simulink model "Fixed_Base_Plant"  (R2026b)
settings: Solver=VariableStepAuto
undefined symbols (not defined in the file): fractalcoef, X, Y, Z
libraries: sm_lib x16, nesl_utility x9, Simulation_Blocks x2, simulink_extras x1, mspsensorlib x1
settings Model: Creator=Janelyn Anderson  LastModifiedBy=Janelyn Anderson

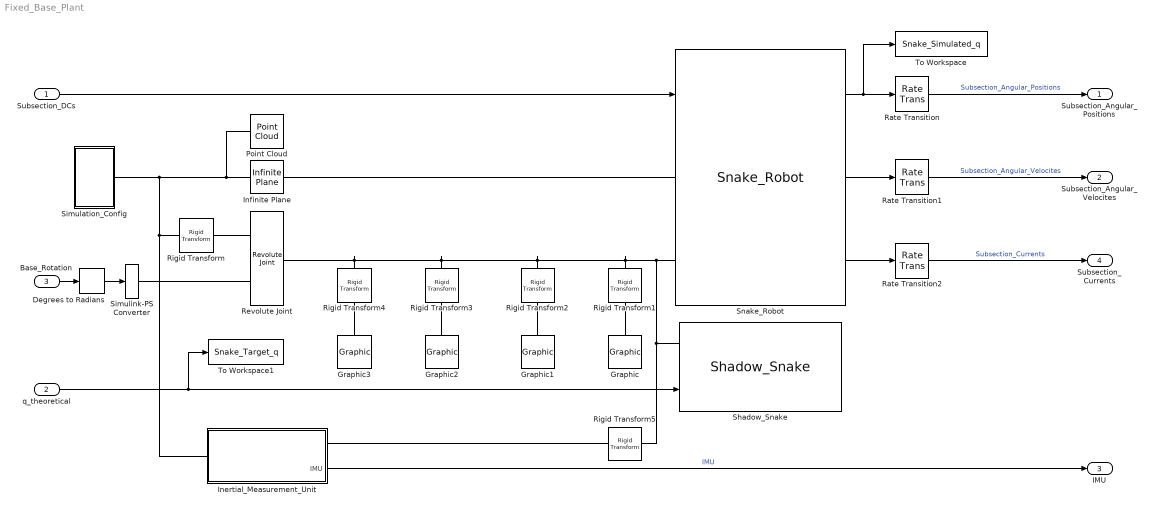
== system Fixed_Base_Plant ==
  Subsection_DCs : Inport
  q_theoretical : Inport  Port=2
  Base_Rotation : Inport  Port=3
  Degrees to Radians : simulink_extras/Transformations/Degrees to Radians
  Graphic : sm_lib/Body Elements/Graphic  GraphicType=Marker  MarkerShape=Sphere  MarkerSize=10  GraphicVisPropType=SimpleVisualProperties  GraphicDiffuseColor=[1 1 0]  GraphicOpacity=1  GraphicSpecularColor=[0.5 0.5 0.5 1.0]  GraphicAmbientColor=[0.15 0.15 0.15 1.0]  GraphicEmissiveColor=[0.0 0.0 0.0 1.0]  GraphicShininess=75
  Graphic1 : sm_lib/Body Elements/Graphic  GraphicType=Marker  MarkerShape=Sphere  MarkerSize=10  GraphicVisPropType=SimpleVisualProperties  GraphicDiffuseColor=[0 1 0]  GraphicOpacity=1  GraphicSpecularColor=[0.5 0.5 0.5 1.0]  GraphicAmbientColor=[0.15 0.15 0.15 1.0]  GraphicEmissiveColor=[0.0 0.0 0.0 1.0]  GraphicShininess=75
  Graphic2 : sm_lib/Body Elements/Graphic  GraphicType=Marker  MarkerShape=Sphere  MarkerSize=10  GraphicVisPropType=SimpleVisualProperties  GraphicDiffuseColor=[1 0 0]  GraphicOpacity=1  GraphicSpecularColor=[0.5 0.5 0.5 1.0]  GraphicAmbientColor=[0.15 0.15 0.15 1.0]  GraphicEmissiveColor=[0.0 0.0 0.0 1.0]  GraphicShininess=75
  Graphic3 : sm_lib/Body Elements/Graphic  GraphicType=Marker  MarkerShape=Sphere  MarkerSize=10  GraphicVisPropType=SimpleVisualProperties  GraphicDiffuseColor=[0 0 1]  GraphicOpacity=1  GraphicSpecularColor=[0.5 0.5 0.5 1.0]  GraphicAmbientColor=[0.15 0.15 0.15 1.0]  GraphicEmissiveColor=[0.0 0.0 0.0 1.0]  GraphicShininess=75
  Inertial_Measurement_Unit : Subsystem
      settings: PortSchema="{\"entries\":[{\"content\":{\"sides\":[{\"content\":{\"connectorIds\":[\"LConn1\"]},\"type\":\"ConnectorPlacement.EquallySpacedRectSide\",\"uuid\":\"83640582-12e8-48aa-a086-d986329aaf09\"},{\"content\":{\"connectorIds\":[\"RConn1\",\"Out1\"],\"side\":\"RIGHT\"},\"type\":\"ConnectorPlacement.EquallySpacedRectSide\",\"uuid\":\"2d285237-615f-43bd-9bcd-fec2f137a93b\"},{\"content\":{\"side\":\"TOP\"},\"type\":\"ConnectorPlacement.EquallySpacedRectSide\",\"uuid\":\"9a803d3e-15ac-4be1-bdbe-8bb20f8175ea\"}]},\"type\":\"ConnectorPlacement.EquallySpacedConnector\",\"uuid\":\"2b15680b-56f3-4ae6-a253-9b33d5e19e84\"}],\"packageUris\":[\"http://schema.mathworks.com/mf0/Connector/R2020b\"],\"version\":\"1.0\"}"
  Infinite Plane : sm_lib/Curves and Surfaces/Infinite Plane  GraphicType=Rectangle  GraphicPlaneWidth=2  GraphicPlaneWidthUnits=m  GraphicPlaneHeight=2  GraphicPlaneHeightUnits=m  GraphicVisPropType=AdvancedVisualProperties  GraphicDiffuseColor=[0.5 0.5 0.5]  GraphicOpacity=1  GraphicSpecularColor=[0.5 0.5 0.5 1.0]  GraphicAmbientColor=[0.15 0.15 0.15 1.0]  GraphicEmissiveColor=[0.0 0.0 0.0 1.0]  GraphicShininess=60
  Point Cloud : sm_lib/Curves and Surfaces/Point Cloud  CoordinatesMatrix=floorGrid  CoordinatesMatrixUnits=m  GraphicType=MarkerCloud  GraphicSphereRadius=1e-2  GraphicSphereRadiusUnits=m  GraphicVisPropType=SimpleVisualProperties  GraphicDiffuseColor=[0.3451 0.3333 0.6863]  GraphicOpacity=0.5  GraphicSpecularColor=[0.5 0.5 0.5 1.0]  GraphicAmbientColor=[0.15 0.15 0.15 1.0]  GraphicEmissiveColor=[0.0 0.0 0.0 1.0]  GraphicShininess=75
  Rate Transition : RateTransition  OutPortSampleTime=1/50
  Rate Transition1 : RateTransition  OutPortSampleTime=1/50
  Rate Transition2 : RateTransition  OutPortSampleTime=1/50
  Revolute Joint : sm_lib/Joints/Revolute Joint  JointMode=Normal  CompositeWrenchDir=FollowerOnBase  CompositeWrenchFrame=BaseFrame  SenseConstraintForce=off  SenseConstraintTorque=off  SenseTotalForce=off  SenseTotalTorque=off  PositionTargetSpecify=off  PositionTargetPriority=High  PositionTargetValue=0  PositionTargetValueUnits=deg  VelocityTargetSpecify=off  VelocityTargetPriority=High  VelocityTargetValue=0  VelocityTargetValueUnits=deg/s  EquilibriumPosition=0  EquilibriumPositionUnits=deg  SpringStiffness=0  SpringStiffnessUnits=N*m/deg  DampingCoefficient=0  DampingCoefficientUnits=N*m/(deg/s)  LowerLimitSpecify=on  LowerLimitBound=-90  LowerLimitBoundUnits=deg  LowerLimitStiffness=1e4  LowerLimitStiffnessUnits=N*m/deg  LowerLimitDamping=10  LowerLimitDampingUnits=N*m/(deg/s)  LowerLimitTransitionRegionWidth=0.1  LowerLimitTransitionRegionWidthUnits=deg  UpperLimitSpecify=on  UpperLimitBound=90  UpperLimitBoundUnits=deg  UpperLimitStiffness=1e4  UpperLimitStiffnessUnits=N*m/deg  UpperLimitDamping=10  UpperLimitDampingUnits=N*m/(deg/s)  UpperLimitTransitionRegionWidth=0.1  UpperLimitTransitionRegionWidthUnits=deg  TorqueActuationMode=ComputedTorque  MotionActuationMode=InputMotion  SensePosition=off  SenseVelocity=off  SenseAcceleration=off  SenseTorqueForce=off  SenseLowerLimitTorqueForce=off  SenseUpperLimitTorqueForce=off
  Rigid Transform : sm_lib/Frames and Transforms/Rigid Transform  RotationMethod=RotationSequence  FollAlignAxisA=+X  BaseAlignAxisA=+Y  FollAlignAxisB=+Y  BaseAlignAxisB=+Z  RotationStandardAxis=+X  RotationAngle=90  RotationAngleUnits=deg  RotationArbitraryAxis=[0 0 1]  RotationSequenceAxes=FollowerAxes  RotationSequence=XZX  RotationSequenceAngles=[90 0 0]  RotationSequenceAnglesUnits=deg  RotationMatrix=[1 0 0;0 1 0;0 0 1]  Quaternion=[1 0 0 0]  TranslationMethod=Cartesian  TranslationCartesianOffset=[0 0 20]  TranslationCartesianOffsetUnits=in  TranslationStandardAxis=+Z  TranslationStandardOffset=0  TranslationStandardOffsetUnits=m  TranslationROffset=0  TranslationROffsetUnits=m  TranslationThetaOffset=0  TranslationThetaOffsetUnits=deg  TranslationZOffset=0  TranslationZOffsetUnits=m
  Rigid Transform1 : sm_lib/Frames and Transforms/Rigid Transform  RotationMethod=StandardAxis  FollAlignAxisA=+X  BaseAlignAxisA=+Y  FollAlignAxisB=+Y  BaseAlignAxisB=+Z  RotationStandardAxis=+Z  RotationAngle=0  RotationAngleUnits=deg  RotationArbitraryAxis=[0 0 1]  RotationSequenceAxes=FollowerAxes  RotationSequence=XYX  RotationSequenceAngles=[0 0 0]  RotationSequenceAnglesUnits=deg  RotationMatrix=[1 0 0;0 1 0;0 0 1]  Quaternion=[1 0 0 0]  TranslationMethod=StandardAxis  TranslationCartesianOffset=[0 0 0]  TranslationCartesianOffsetUnits=m  TranslationStandardAxis=-X  TranslationStandardOffset=1.5  TranslationStandardOffsetUnits=ft  TranslationROffset=0  TranslationROffsetUnits=m  TranslationThetaOffset=0  TranslationThetaOffsetUnits=deg  TranslationZOffset=0  TranslationZOffsetUnits=m
  Rigid Transform2 : sm_lib/Frames and Transforms/Rigid Transform  RotationMethod=StandardAxis  FollAlignAxisA=+X  BaseAlignAxisA=+Y  FollAlignAxisB=+Y  BaseAlignAxisB=+Z  RotationStandardAxis=+Z  RotationAngle=90  RotationAngleUnits=deg  RotationArbitraryAxis=[0 0 1]  RotationSequenceAxes=FollowerAxes  RotationSequence=XYX  RotationSequenceAngles=[0 0 0]  RotationSequenceAnglesUnits=deg  RotationMatrix=[1 0 0;0 1 0;0 0 1]  Quaternion=[1 0 0 0]  TranslationMethod=StandardAxis  TranslationCartesianOffset=[0 0 0]  TranslationCartesianOffsetUnits=m  TranslationStandardAxis=-Y  TranslationStandardOffset=1.5  TranslationStandardOffsetUnits=ft  TranslationROffset=0  TranslationROffsetUnits=m  TranslationThetaOffset=0  TranslationThetaOffsetUnits=deg  TranslationZOffset=0  TranslationZOffsetUnits=m
  Rigid Transform3 : sm_lib/Frames and Transforms/Rigid Transform  RotationMethod=None  FollAlignAxisA=+X  BaseAlignAxisA=+Y  FollAlignAxisB=+Y  BaseAlignAxisB=+Z  RotationStandardAxis=+Z  RotationAngle=180  RotationAngleUnits=deg  RotationArbitraryAxis=[0 0 1]  RotationSequenceAxes=FollowerAxes  RotationSequence=XYX  RotationSequenceAngles=[0 0 0]  RotationSequenceAnglesUnits=deg  RotationMatrix=[1 0 0;0 1 0;0 0 1]  Quaternion=[1 0 0 0]  TranslationMethod=StandardAxis  TranslationCartesianOffset=[0 0 0]  TranslationCartesianOffsetUnits=m  TranslationStandardAxis=+X  TranslationStandardOffset=1.5  TranslationStandardOffsetUnits=ft  TranslationROffset=0  TranslationROffsetUnits=m  TranslationThetaOffset=0  TranslationThetaOffsetUnits=deg  TranslationZOffset=0  TranslationZOffsetUnits=m
  Rigid Transform4 : sm_lib/Frames and Transforms/Rigid Transform  RotationMethod=None  FollAlignAxisA=+X  BaseAlignAxisA=+Y  FollAlignAxisB=+Y  BaseAlignAxisB=+Z  RotationStandardAxis=+Z  RotationAngle=270  RotationAngleUnits=deg  RotationArbitraryAxis=[0 0 1]  RotationSequenceAxes=FollowerAxes  RotationSequence=XYX  RotationSequenceAngles=[0 0 0]  RotationSequenceAnglesUnits=deg  RotationMatrix=[1 0 0;0 1 0;0 0 1]  Quaternion=[1 0 0 0]  TranslationMethod=StandardAxis  TranslationCartesianOffset=[0 0 0]  TranslationCartesianOffsetUnits=m  TranslationStandardAxis=+Y  TranslationStandardOffset=1.5  TranslationStandardOffsetUnits=ft  TranslationROffset=0  TranslationROffsetUnits=m  TranslationThetaOffset=0  TranslationThetaOffsetUnits=deg  TranslationZOffset=0  TranslationZOffsetUnits=m
  Rigid Transform5 : sm_lib/Frames and Transforms/Rigid Transform  RotationMethod=RotationSequence  FollAlignAxisA=+X  BaseAlignAxisA=+Y  FollAlignAxisB=+Y  BaseAlignAxisB=+Z  RotationStandardAxis=+X  RotationAngle=90  RotationAngleUnits=deg  RotationArbitraryAxis=[0 0 1]  RotationSequenceAxes=FollowerAxes  RotationSequence=XZX  RotationSequenceAngles=[-90 0 0]  RotationSequenceAnglesUnits=deg  RotationMatrix=[1 0 0;0 1 0;0 0 1]  Quaternion=[1 0 0 0]  TranslationMethod=None  TranslationCartesianOffset=[0 0 20]  TranslationCartesianOffsetUnits=in  TranslationStandardAxis=+Z  TranslationStandardOffset=0  TranslationStandardOffsetUnits=m  TranslationROffset=0  TranslationROffsetUnits=m  TranslationThetaOffset=0  TranslationThetaOffsetUnits=deg  TranslationZOffset=0  TranslationZOffsetUnits=m
  Shadow_Snake : Simulation_Blocks/Shadow_Snake  SystemSampleTime=-1  VariantActivationTime=update diagram  EmptyChoice=off  PassThrough=off  PassThroughVariantControl=(default)  EmptyChoiceVariantControl=(default)  AllowFlexibleInterface=on  Latency=0  AutoFrameSizeCalculation=off
      settings: PortSchema="{\"entries\":[{\"content\":{\"sides\":[{\"content\":{\"connectorIds\":[\"LConn1\",\"In1\"]},\"type\":\"ConnectorPlacement.EquallySpacedRectSide\",\"uuid\":\"1314429c-2aac-4de2-891a-5a96a4d19acb\"},{\"content\":{\"side\":\"RIGHT\"},\"type\":\"ConnectorPlacement.EquallySpacedRectSide\",\"uuid\":\"25d2558a-3032-4dee-ac42-109954eda9a9\"},{\"content\":{\"side\":\"TOP\"},\"type\":\"ConnectorPlacement.EquallySpacedRectSide\",\"uuid\":\"581d579a-08be-4756-9415-fbb6b4806955\"}]},\"type\":\"ConnectorPlacement.EquallySpacedConnector\",\"uuid\":\"048d360f-47b2-4b65-b276-ef94c0e4ed46\"}],\"packageUris\":[\"http://schema.mathworks.com/mf0/Connector/R2020b\"],\"version\":\"1.0\"}"
  Simulation_Config : Subsystem
  Simulink-PS Converter : nesl_utility/Simulink-PS Converter  PhysicalDomain=network_engine_domain  SubClassName=ps_input  LeftPortType=input  RightPortType=output  PseudoPeriodic=off  Frequencies=[]  NoiseDistribution=none  NoiseParameters=[]  Unit=1  AffineConversion=off  FilteringAndDerivatives=filter  SimscapeFilterOrder=2  InputFilterTimeConstant=0.001  UdotUserProvided=0
  Snake_Robot : Simulation_Blocks/Snake_Robot  SystemSampleTime=-1  VariantActivationTime=update diagram  EmptyChoice=off  PassThrough=off  PassThroughVariantControl=(default)  EmptyChoiceVariantControl=(default)  AllowFlexibleInterface=on  Latency=0  AutoFrameSizeCalculation=off
  To Workspace : ToWorkspace  VariableName=Snake_Simulated_q  SaveFormat=Timeseries  SampleTime=1/30
  To Workspace1 : ToWorkspace  VariableName=Snake_Target_q  SaveFormat=Timeseries  SampleTime=1/30
  Subsection_Angular_Positions : Outport
  Subsection_Angular_Velocites : Outport  Port=2
  IMU : Outport  Port=3
  Subsection_Currents : Outport  Port=4
  wires:
  Snake_Robot/1 -> Rate Transition/1, To Workspace/1
  Snake_Robot/2 -> Rate Transition1/1
  Snake_Robot/3 -> Rate Transition2/1
  Subsection_DCs/1 -> Snake_Robot/1
  Rate Transition/1 -> Subsection_Angular_Positions/1  "Subsection_Angular_Positions"
  Rate Transition2/1 -> Subsection_Currents/1  "Subsection_Currents"
  Inertial_Measurement_Unit/1(IMU) -> IMU/1  "IMU"
  q_theoretical/1 -> To Workspace1/1, Shadow_Snake/1
  Rate Transition1/1 -> Subsection_Angular_Velocites/1  "Subsection_Angular_Velocites"
  Base_Rotation/1 -> Degrees to Radians/1
  Degrees to Radians/1 -> Simulink-PS Converter/1
  connections:
  Rigid Transform5/LConn1 -- Shadow_Snake/LConn1 -- Snake_Robot/LConn2 -- Rigid Transform4/LConn1 -- Revolute Joint/RConn1 -- Rigid Transform3/LConn1 -- Rigid Transform2/LConn1 -- Rigid Transform1/LConn1
  Point Cloud/LConn1 -- Simulation_Config/RConn1 -- Rigid Transform/LConn1 -- Inertial_Measurement_Unit/LConn1 -- Infinite Plane/LConn1
  Infinite Plane/RConn1 -- Snake_Robot/LConn1
  Revolute Joint/LConn1 -- Rigid Transform/RConn1
  Simulink-PS Converter/RConn1 -- Revolute Joint/LConn2
  Rigid Transform1/RConn1 -- Graphic/RConn1
  Rigid Transform2/RConn1 -- Graphic1/RConn1
  Rigid Transform3/RConn1 -- Graphic2/RConn1
  Rigid Transform4/RConn1 -- Graphic3/RConn1
  Rigid Transform5/RConn1 -- Inertial_Measurement_Unit/RConn1

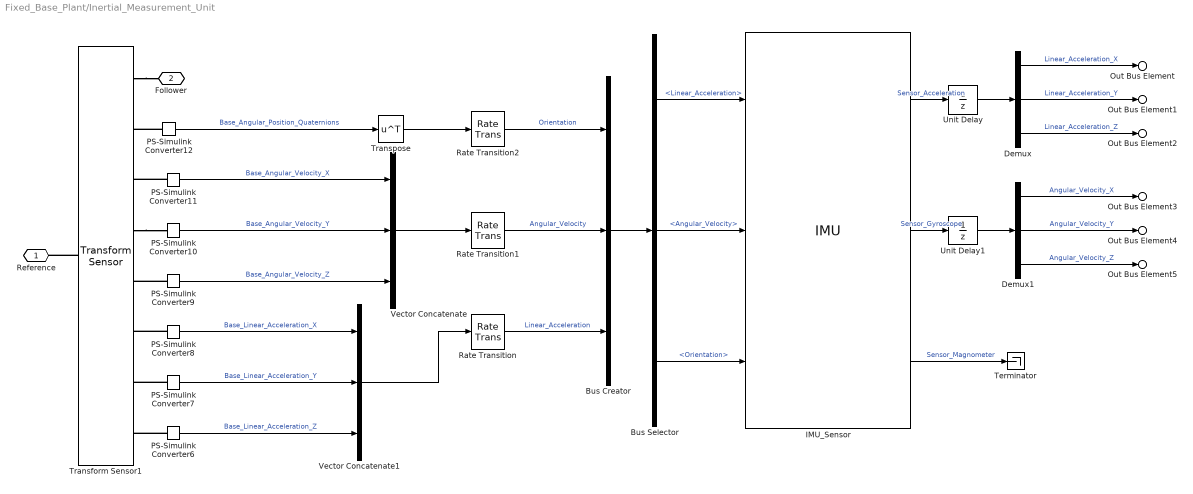
== system Fixed_Base_Plant/Inertial_Measurement_Unit ==
  Bus Creator : BusCreator  Inputs=3
  Bus Selector : BusSelector  OutputSignals=Linear_Acceleration,Angular_Velocity,Orientation
  Demux : Demux  Outputs=3
  Demux1 : Demux  Outputs=3
  IMU_Sensor : mspsensorlib/IMU  DispRefFrame=NED  TemperaturePort=off  Temperature=25  MagneticFieldPort=off  MagneticFieldNED=[ 27.5550, -2.4169, -16.0849 ]  MagneticFieldENU=[ -2.4169, 27.5550, 16.0849 ]  SeedDouble=67  SimulateUsing=Code generation  AccelParamsMeasurementRange=Inf  AccelParamsResolution=0  AccelParamsConstantBias=[ 0, 0, 0 ]  AccelParamsAxesMisalignment=[ 100, 0, 0; 0, 100, 0; 0, 0, 100 ]  AccelParamsNoiseDensity=[ 0, 0, 0 ]  AccelParamsBiasInstability=[ 0, 0, 0 ]  AccelParamsBiasInstabilityNumerator=fractalcoef().Numerator  AccelParamsBiasInstabilityDenominator=fractalcoef().Denominator  AccelParamsRandomWalk=[ 0, 0, 0 ]  AccelParamsNoiseType=double-sided  AccelParamsTemperatureBias=[ 0, 0, 0 ]  AccelParamsTemperatureScaleFactor=[ 0, 0, 0 ]  GyroParamsMeasurementRange=Inf  GyroParamsResolution=0  GyroParamsConstantBias=[ 0, 0, 0 ]  GyroParamsAxesMisalignment=[ 100, 0, 0; 0, 100, 0; 0, 0, 100 ]  GyroParamsAccelerationBias=[ 0, 0, 0 ]  GyroParamsNoiseDensity=[ 0, 0, 0 ]  GyroParamsBiasInstability=[ 0, 0, 0 ]  GyroParamsBiasInstabilityNumerator=fractalcoef().Numerator  GyroParamsBiasInstabilityDenominator=fractalcoef().Denominator  GyroParamsRandomWalk=[ 0, 0, 0 ]  GyroParamsNoiseType=double-sided  GyroParamsTemperatureBias=[ 0, 0, 0 ]  GyroParamsTemperatureScaleFactor=[ 0, 0, 0 ]  MagParamsMeasurementRange=Inf  MagParamsResolution=0  MagParamsConstantBias=[ 0, 0, 0 ]  MagParamsAxesMisalignment=[ 100, 0, 0; 0, 100, 0; 0, 0, 100 ]  MagParamsNoiseDensity=[ 0, 0, 0 ]  MagParamsBiasInstability=[ 0, 0, 0 ]  MagParamsBiasInstabilityNumerator=fractalcoef().Numerator  MagParamsBiasInstabilityDenominator=fractalcoef().Denominator  MagParamsRandomWalk=[ 0, 0, 0 ]  MagParamsNoiseType=double-sided  MagParamsTemperatureBias=[ 0, 0, 0 ]  MagParamsTemperatureScaleFactor=[ 0, 0, 0 ]
  PS-Simulink Converter{6..12} (7 alike) : nesl_utility/PS-Simulink Converter  PhysicalDomain=network_engine_domain  SubClassName=ps_output  LeftPortType=input  RightPortType=output  PseudoPeriodic=off  Frequencies=[]  VectorFormat=inherit  Unit=inherit  AffineConversion=off
  Rate Transition : RateTransition  OutPortSampleTime=t_s
  Rate Transition1 : RateTransition  OutPortSampleTime=t_s
  Rate Transition2 : RateTransition  OutPortSampleTime=t_s
  Terminator : Terminator
  Transform Sensor1 : sm_lib/Frames and Transforms/Transform Sensor  ObservationFrame=World  ExpressedInFrame=World  RotationSequence=XYX  SenseAngle=off  SenseAxis=off  SenseQ=on  SenseR=off  SenseRotationSequence=off  SenseOmegaX=on  SenseOmegaY=on  SenseOmegaZ=on  SenseOmega=off  SenseQDot=off  SenseRDot=off  SenseRotationSequenceDot=off  SenseAlphaX=off  SenseAlphaY=off  SenseAlphaZ=off  SenseAlpha=off  SenseQDDot=off  SenseRDDot=off  SenseX=off  SenseY=off  SenseZ=off  SenseXYZ=off  SenseRad=off  SenseAzim=off  SenseDist=off  SenseInc=off  SenseXDot=off  SenseYDot=off  SenseZDot=off  SenseXYZDot=off  SenseRadDot=off  SenseAzimDot=off  SenseDistDot=off  SenseIncDot=off  SenseXDDot=on  SenseYDDot=on  SenseZDDot=on  SenseXYZDDot=off  SenseRadDDot=off  SenseAzimDDot=off  SenseDistDDot=off  SenseIncDDot=off
  Transpose : Math  Operator=transpose
  Unit Delay : UnitDelay  SampleTime=-1
  Unit Delay1 : UnitDelay  SampleTime=-1
  Vector Concatenate : Concatenate  NumInputs=3  Mode=Multidimensional array  ConcatenateDimension=2
  Vector Concatenate1 : Concatenate  NumInputs=3  Mode=Multidimensional array  ConcatenateDimension=2
  Reference : PMIOPort  Side=Left
  Follower : PMIOPort  Port=2  Side=Right
  Out Bus Element : Outport  PortName=IMU  Element=Linear_Accleration.Linear_Acceleration_X
  Out Bus Element1 : Outport  PortName=IMU  Element=Linear_Accleration.Linear_Acceleration_Y
  Out Bus Element2 : Outport  PortName=IMU  Element=Linear_Accleration.Linear_Acceleration_Z
  Out Bus Element3 : Outport  PortName=IMU  Element=Angular_Velocity.Angular_Velocity_X
  Out Bus Element4 : Outport  PortName=IMU  Element=Angular_Velocity.Angular_Velocity_Y
  Out Bus Element5 : Outport  PortName=IMU  Element=Angular_Velocity.Angular_Velocity_Z
  wires:
  Unit Delay1/1 -> Demux1/1
  Unit Delay/1 -> Demux/1
  PS-Simulink Converter11/1 -> Vector Concatenate/1  "Base_Angular_Velocity_X"
  PS-Simulink Converter12/1 -> Transpose/1  "Base_Angular_Position_Quaternions"
  PS-Simulink Converter10/1 -> Vector Concatenate/2  "Base_Angular_Velocity_Y"
  PS-Simulink Converter7/1 -> Vector Concatenate1/2  "Base_Linear_Acceleration_Y"
  PS-Simulink Converter8/1 -> Vector Concatenate1/1  "Base_Linear_Acceleration_X"
  PS-Simulink Converter6/1 -> Vector Concatenate1/3  "Base_Linear_Acceleration_Z"
  PS-Simulink Converter9/1 -> Vector Concatenate/3  "Base_Angular_Velocity_Z"
  Transpose/1 -> Rate Transition2/1
  Vector Concatenate/1 -> Rate Transition1/1
  Vector Concatenate1/1 -> Rate Transition/1
  Bus Creator/1 -> Bus Selector/1
  Rate Transition/1 -> Bus Creator/3  "Linear_Acceleration"
  Rate Transition1/1 -> Bus Creator/2  "Angular_Velocity"
  Rate Transition2/1 -> Bus Creator/1  "Orientation"
  Bus Selector/3 -> IMU_Sensor/3  "<Orientation>"
  Bus Selector/2 -> IMU_Sensor/2  "<Angular_Velocity>"
  Bus Selector/1 -> IMU_Sensor/1  "<Linear_Acceleration>"
  IMU_Sensor/1 -> Unit Delay/1  "Sensor_Acceleration"
  IMU_Sensor/2 -> Unit Delay1/1  "Sensor_Gyroscope"
  IMU_Sensor/3 -> Terminator/1  "Sensor_Magnometer"
  Demux/1 -> Out Bus Element/1  "Linear_Acceleration_X"
  Demux/2 -> Out Bus Element1/1  "Linear_Acceleration_Y"
  Demux/3 -> Out Bus Element2/1  "Linear_Acceleration_Z"
  Demux1/1 -> Out Bus Element3/1  "Angular_Velocity_X"
  Demux1/2 -> Out Bus Element4/1  "Angular_Velocity_Y"
  Demux1/3 -> Out Bus Element5/1  "Angular_Velocity_Z"
  connections:
  Transform Sensor1/LConn1 -- Reference/RConn1
  Transform Sensor1/RConn1 -- Follower/RConn1
  PS-Simulink Converter12/LConn1 -- Transform Sensor1/RConn2
  PS-Simulink Converter11/LConn1 -- Transform Sensor1/RConn3
  Transform Sensor1/RConn4 -- PS-Simulink Converter10/LConn1
  PS-Simulink Converter9/LConn1 -- Transform Sensor1/RConn5
  PS-Simulink Converter8/LConn1 -- Transform Sensor1/RConn6
  PS-Simulink Converter7/LConn1 -- Transform Sensor1/RConn7
  PS-Simulink Converter6/LConn1 -- Transform Sensor1/RConn8

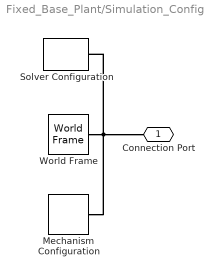
== system Fixed_Base_Plant/Simulation_Config ==
  Mechanism Configuration : sm_lib/Utilities/Mechanism Configuration  UniformGravity=Constant  GravityVector=[0 0 -9.81]  GravityVectorUnits=m/s^2  LinearizationDelta=0.001  JointModeTransitionNonlinearIterations=2
  Solver Configuration : nesl_utility/Solver Configuration  PhysicalDomain=network_engine_domain  SubClassName=solver  LeftPortType=input  RightPortType=generic  Tones=[]  Harmonics=[]  SimulateNoise=off  Profile=off  UseLocalSampling=off  EnableSwitchedLinearOptims=on  FrequencyDomain=off  UseCCode=off  RelTol=0.001  AbsTol=0.001  MinStep=1e-09  ToWorkspace=off  RevertToSquareIcSolve=off  NumHomotopyIterations=100  PhasorMode=off  PhasorModeNumHarmonics=1  ConsistencySolver=NEWTON_XTOL_AFTER_FTOL  CanonicalOrdering=CANONICAL  OptimizeIntermediates=OPTIMIZED  MulticoreSolverChoice=BACKWARD_EULER  IndexReductionMethod=DerivativeReplacement  DoDC=off  ResidualTolerance=1e-09  ConsistencyTolSource=GLOBAL  ConsistencyAbsTol=0.001  ConsistencyRelTol=0.001  ConsistencyTolFactor=0.001  UseLocalSolver=off  LocalSolverChoice=NE_BACKWARD_EULER_ADVANCER  ResolveIndetEquations=on  FunctionEvalNumThread=1  LocalSolverSampleTime=0.001  DoFixedCost=off  MaxNonlinIter=3  MaxModeIter=2  ComputeImpulses=off  ImpulseIterations=2  LinearAlgebra=auto  LinearAlgebraNumThread=0  EquationFormulation=NE_TIME_EF  DelaysMemoryBudget=1024  AutomaticFiltering=on  FilteringTimeConstant=0.001  PartitionStorageMethod=AS_NEEDED  PartitionMemoryBudget=1024  PartitionMethod=BALANCED  MultibodyUseLocalSolver=off  MultibodyLocalSolverChoice=ODE1  MultibodyLocalSolverSampleTime=0.001
  World Frame : sm_lib/Frames and Transforms/World Frame
  Connection Port : PMIOPort  Side=Right
  connections:
  Mechanism Configuration/RConn1 -- Solver Configuration/RConn1 -- World Frame/RConn1 -- Connection Port/RConn1
